simulink model "Q1c_VF_PI"  (R2024b)
settings: Solver=VariableStepAuto  StartTime=0.0  StopTime=5  RelTol=1e-3
model workspace (MAT data in the model file):
  TL = 10
libraries: spsAsynchronousMachineSIUnitsLib x1, spsDCVoltageSourceLib x1, eePwmGeneratorTwoLevel x1, spsUniversalBridgeLib x1, sps_lib x1
settings Model: Creator=mehme  LastModifiedBy=mehme

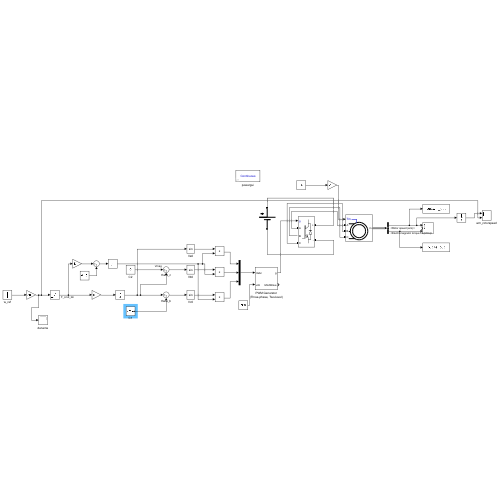
[thumbnail: Simulink's stored preview of the top-level diagram]
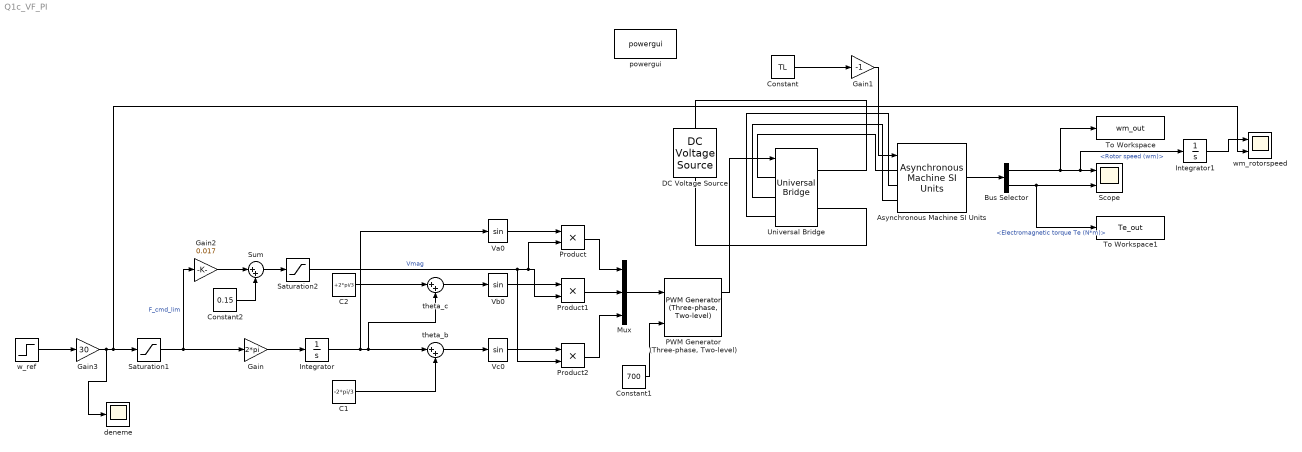
== system Q1c_VF_PI ==
  Asynchronous Machine SI Units : spsAsynchronousMachineSIUnitsLib/Asynchronous Machine SI Units  RotorType=Squirrel-cage  PresetModel=No  MechanicalLoad=Torque Tm  ShowDetailedParameters=on  ReferenceFrame=Rotor  Units=SI  MeasurementBus=off  NominalParameters=[1.845e+04 400 50]  VoltageRatio=1  Stator=[0.5968 0.0003495]  Rotor=[0.6258 0.005473]  Cage1=[0.4155 0.002066]  Cage2=[0.4168 0.0003495]  Lm=0.0354  Mechanical=[0.05 0.005879 2]  PolePairs=2  InitialConditions=[0 0 0 0 0 0 0 0]  SimulateSaturation=off  Saturation=[14.03593122, 27.81365428, 53.79336849, 72.68890987, 97.98006896, 148.6815601, 215.7428561, 302.9841135, 428.7778367 ; 230, 322, 414, 460, 506, 552, 598, 644, 690]  LoadFlowParameters=1492000  TsPowergui=0  TsBlock=-1  IterativeModel=Trapezoidal non iterative  IterativeDiscreteModel=Trapezoidal non iterative  Pmec=1.492e+006
  Bus Selector : BusSelector  OutputSignals=Mechanical.Rotor speed (wm),Mechanical.Electromagnetic torque Te (N*m)
  C1 : Constant  Value=-2*pi/3
  C2 : Constant  Value=+2*pi/3
  Constant : Constant  Value=TL  SampleTime=0
  Constant1 : Constant  Value=700
  Constant2 : Constant  Value=0.15
  DC Voltage Source : spsDCVoltageSourceLib/DC Voltage Source  Amplitude=700  Measurements=Voltage
  Gain : Gain  Gain=2*pi
  Gain1 : Gain  Gain=-1
  Gain2 : Gain  Gain=0.017
  Gain3 : Gain  Gain=30
  Integrator : Integrator
  Integrator1 : Integrator
  Mux : Mux  Inputs=3
  "PWM Generator (Three-phase, Two-level)" : eePwmGeneratorTwoLevel/PWM Generator (Three-phase, Two-level)  PWMMode=Continuous PWM (CPWM)  CPWMMode=SPWM: sinusoidal PWM  DPWMMode=60 DPWM: 60 degree discontinuous PWM  fsw=1e3  Ts=5e-5
      settings: LibrarySourceBlock=|
      | ee_sl_lib/Pulse Width
      | Modulation/PWM Generator
      | (Three-phase, Two-level)
  Product : Product
  Product1 : Product
  Product2 : Product
  Saturation1 : Saturate  UpperLimit=50  LowerLimit=0
  Saturation2 : Saturate  UpperLimit=1  LowerLimit=0
  Scope : Scope  NumInputPorts=3
  Sum : Sum  Inputs=|++
  To Workspace : ToWorkspace  VariableName=wm_out  SaveFormat=Timeseries  SampleTime=-1
  To Workspace1 : ToWorkspace  VariableName=Te_out  SaveFormat=Timeseries  SampleTime=-1
  Universal Bridge : spsUniversalBridgeLib/Universal Bridge  Arms=3  SnubberResistance=1e5  SnubberCapacitance=Inf  Device=IGBT / Diodes  Ron=1e-3  Lon=0  ForwardVoltages="[  0  0  ]"  ForwardVoltage=0  GTOparameters=[ 10e-6 , 20e-6 ]  IGBTparameters=[ 1e-6 , 2e-6 ]  Measurements=None  Measurements_2=None  converterType=Rectifier
  Va0 : Trigonometry
  Vb0 : Trigonometry
  Vc0 : Trigonometry
  deneme : Scope
  powergui : sps_lib/powergui  Priority=1  SimulationMode=Continuous  SampleTime=50e-6  frequency=60  Iterations=50  frequencyindice=50  Pbase=100e6  ErrMax=1e-4  UnitsV=kV  UnitsW=MW  buscounter=0  FunctionMessages=off  echomessages=off  EnableUseOfTLC=off  CurrentSourceSwitches=on  DisableSnubberDevices=off  DisableRonSwitches=off  DisableVfSwitches=off  DisplayEquations=off  AutomaticDiscreteSolvers=off  SolverType=Tustin/Backward Euler (TBE)  Interpol=off  ExternalGateDelay=off  methode=off  Ts=100  x0status=blocks  SPID=on  SwTol=0  HookPort=off  NonlinearTolerance=1e-4  nMaxIteration=100  ContinueOnMaxIteration=off  RestoreLinks=warning  ResistiveCurrentMeasurement=off  Frange=[0:2:500]  Ylog=off  Xlog=on  ShowGrid=off  save=off  variable=ZData  structure=0  ZoomFFT=off  StartTime=0.0  cycles=1  DisplayStyle=1  fundamental=60  FreqAxis=off  MaxFrequency=1000  frequencyindicesteady=1  RmsSteady=1  display=off
  theta_b : Sum  Inputs=|++
  theta_c : Sum  Inputs=|++
  w_ref : Step  Time=0.4  After=1600  SampleTime=0
  wm_rotorspeed : Scope  NumInputPorts=2
  wires:
  Asynchronous Machine SI Units/1 -> Bus Selector/1
  Bus Selector/1 -> To Workspace/1, Integrator1/1, Scope/1  "<Rotor speed (wm)>"
  Bus Selector/2 -> Scope/3, To Workspace1/1  "<Electromagnetic torque Te (N*m)>"
  "PWM Generator (Three-phase, Two-level)"/1 -> Universal Bridge/1
  Constant1/1 -> "PWM Generator (Three-phase, Two-level)"/2
  Gain/1 -> Integrator/1
  Integrator/1 -> Va0/1, theta_c/2, theta_b/1
  C1/1 -> theta_b/2
  C2/1 -> theta_c/1
  theta_b/1 -> Vc0/1
  theta_c/1 -> Vb0/1
  Va0/1 -> Product/1
  Vc0/1 -> Product2/1
  Vb0/1 -> Product1/1
  Product/1 -> Mux/1
  Product1/1 -> Mux/2
  Product2/1 -> Mux/3
  Mux/1 -> "PWM Generator (Three-phase, Two-level)"/1
  Gain2/1 -> Sum/1
  Constant2/1 -> Sum/2
  Sum/1 -> Saturation2/1
  Saturation2/1 -> Product2/2, Product/2, Product1/2  "Vmag"
  Constant/1 -> Gain1/1
  Gain1/1 -> Asynchronous Machine SI Units/1
  Saturation1/1 -> Gain/1, Gain2/1  "F_cmd_lim"
  w_ref/1 -> Gain3/1
  Gain3/1 -> deneme/1, wm_rotorspeed/2, Saturation1/1
  Integrator1/1 -> wm_rotorspeed/1
  connections:
  DC Voltage Source/LConn1 -- Universal Bridge/RConn2
  DC Voltage Source/RConn1 -- Universal Bridge/RConn1
  Universal Bridge/LConn1 -- Asynchronous Machine SI Units/LConn1
  Universal Bridge/LConn2 -- Asynchronous Machine SI Units/LConn3
  Universal Bridge/LConn3 -- Asynchronous Machine SI Units/LConn2
